simulink model "Physics_Testing"  (R2025b)
settings: Solver=VariableStepAuto  StartTime=0.0  StopTime=10.0  RelTol=1e-3
settings Model: Creator=Admin  LastModifiedBy=Admin

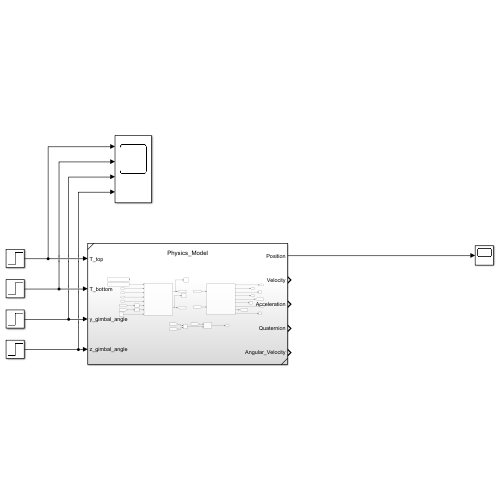
[thumbnail: Simulink's stored preview of the top-level diagram]
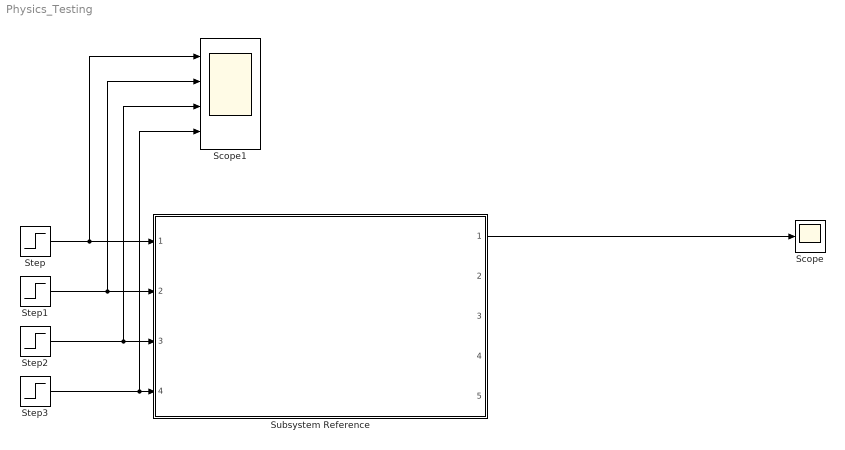
== system Physics_Testing ==
  Scope : Scope
      settings: ActiveDisplayYMinimum=-1  ActiveDisplayYMaximum=1
  Scope1 : Scope  NumInputPorts=4
      settings: ActiveDisplayYMinimum=-1  ActiveDisplayYMaximum=1
  Step : Step  SampleTime=0
  Step1 : Step  SampleTime=0
  Step2 : Step  After=0  SampleTime=0
  Step3 : Step  After=0  SampleTime=0
  Subsystem Reference : Subsystem  ReferencedSubsystem=Physics_Model
  wires:
  Step3/1 -> Scope1/4, Subsystem Reference/4
  Step2/1 -> Scope1/3, Subsystem Reference/3
  Subsystem Reference/1 -> Scope/1
  Step1/1 -> Scope1/2, Subsystem Reference/2
  Step/1 -> Subsystem Reference/1, Scope1/1
